simulink model "current_controller_Buck_converter_A01"  (R2025b)
settings: Solver=ode15s  StartTime=0.0  StopTime=0.1  FixedStep=Ts  RelTol=1e-3
values from neighbouring files (symbols this model uses):
  H = -1/(s*R*C)    [type_1_compansator_A01.m]
  R_f = 0.2    [buck_converter_parameters_A01.m]
undefined symbols (not defined in the file or in its folder): ma, Ts
libraries: spsSeriesRLCBranchLib x3, spsCurrentMeasurementLib x2, cstblocks x1, simulink x1, spsDCVoltageSourceLib x1, spsDiodeLib x1, spsMosfetLib x1, spsVoltageMeasurementLib x1, sps_lib x1
settings Model: Creator=arif  LastModifiedBy=arif
settings SolverCC: ZeroCrossAlgorithm=Adaptive
settings DebuggingCC: MaskedZcDiagnostic=none  IgnoredZcDiagnostic=none

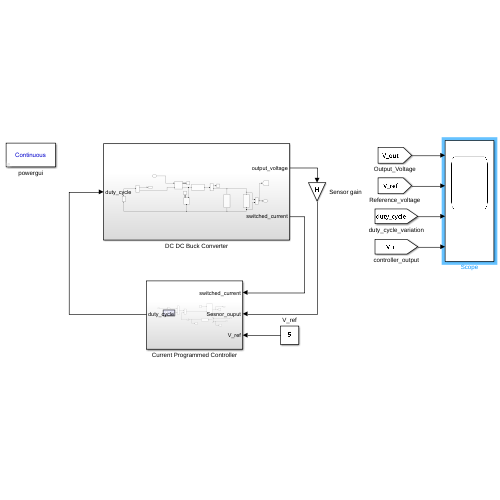
[thumbnail: Simulink's stored preview of the top-level diagram]
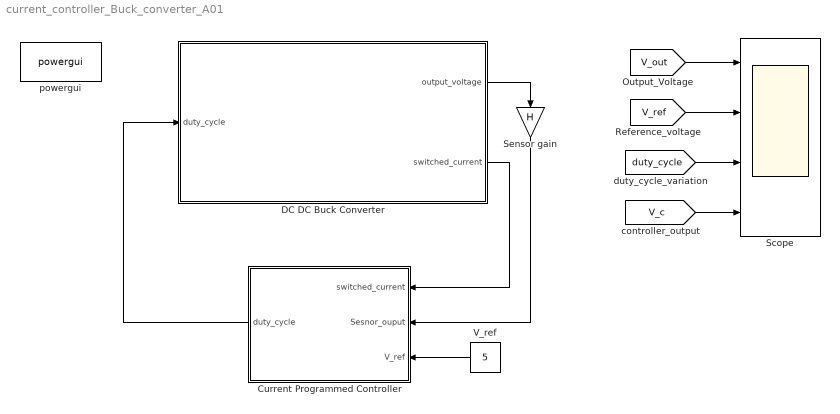
== system current_controller_Buck_converter_A01 ==
  Current Programmed Controller : Subsystem
      settings: PortSchema="{\"entries\":[{\"content\":{\"sides\":[{\"content\":{\"connectorIds\":[\"Out1\"]},\"type\":\"ConnectorPlacement.EquallySpacedRectSide\",\"uuid\":\"f14b5529-64c8-475c-92f8-e2614ee0a8ad\"},{\"content\":{\"connectorIds\":[\"In1\",\"In2\",\"In3\"],\"side\":\"RIGHT\"},\"type\":\"ConnectorPlacement.EquallySpacedRectSide\",\"uuid\":\"ccab92c4-01d4-490c-899e-0d4eb02db195\"},{\"content\":{\"side\":\"TOP\"},\"type\":\"ConnectorPlacement.EquallySpacedRectSide\",\"uuid\":\"b1180856-4250-44ce-8479-d48f19e18262\"}]},\"type\":\"ConnectorPlacement.EquallySpacedConnector\",\"uuid\":\"9f0b6857-1f65-4299-9855-6d8c8b04cf8e\"}],\"packageUris\":[\"http://schema.mathworks.com/mf0/Connector/R2020b\"],\"version\":\"1.0\"}"
  DC DC Buck Converter : Subsystem
  Scope : Scope  NumInputPorts=4
      settings: ActiveDisplayYMinimum=-4.2219957385816729  ActiveDisplayYMaximum=38.006361395242614
  Sensor gain : Gain  Gain=H
  V_ref : Constant  Value=5
  powergui : sps_lib/powergui  Priority=1  SimulationMode=Continuous  SampleTime=50e-6  frequency=60  Iterations=50  frequencyindice=0  Pbase=100e6  ErrMax=1e-4  UnitsV=kV  UnitsW=MW  buscounter=0  FunctionMessages=off  echomessages=off  EnableUseOfTLC=off  CurrentSourceSwitches=off  DisableSnubberDevices=off  DisableRonSwitches=off  DisableVfSwitches=off  DisplayEquations=off  AutomaticDiscreteSolvers=off  SolverType=Tustin/Backward Euler (TBE)  Interpol=off  ExternalGateDelay=off  methode=off  Ts=100  x0status=blocks  SPID=on  SwTol=0  HookPort=off  NonlinearTolerance=1e-4  nMaxIteration=100  ContinueOnMaxIteration=off  RestoreLinks=warning  ResistiveCurrentMeasurement=off  Frange=[0:2:500]  Ylog=off  Xlog=on  ShowGrid=off  save=off  variable=ZData  structure=0  ZoomFFT=off  StartTime=0.0  cycles=1  DisplayStyle=1  fundamental=60  FreqAxis=off  MaxFrequency=1000  frequencyindicesteady=1  RmsSteady=1  display=off
  wires:
  [V_c] -> Scope/4
  [duty_cycle] -> Scope/3
  [V_out] -> Scope/1
  [V_ref] -> Scope/2
  V_ref/1 -> Current Programmed Controller/3(V_ref)
  DC DC Buck Converter/1(output_voltage) -> Sensor gain/1
  Current Programmed Controller/1(duty_cycle) -> DC DC Buck Converter/1(duty_cycle)
  DC DC Buck Converter/2(switched_current) -> Current Programmed Controller/1(switched_current)
  Sensor gain/1 -> Current Programmed Controller/2(Sesnor_ouput)

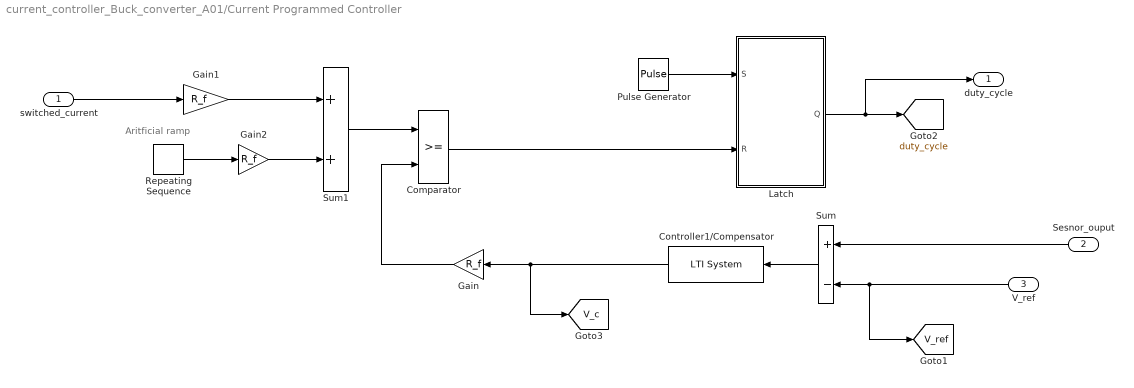
== system current_controller_Buck_converter_A01/Current Programmed Controller ==
  note: Aritficial ramp
  switched_current : Inport
  Sesnor_ouput : Inport  Port=2
  V_ref : Inport  Port=3
  Comparator : RelationalOperator  OutDataTypeStr=boolean  RndMeth=Simplest  InputSameDT=off
  Controller1/Compensator : cstblocks/LTI System  sys=G_PI  IC=[]  PadeOrder=0
  Gain : Gain  Gain=R_f
  Gain1 : Gain  Gain=R_f
  Gain2 : Gain  Gain=R_f
  Latch : Subsystem
  Pulse Generator : DiscretePulseGenerator  PulseType=Time based  Period=Ts  PulseWidth=99
  Repeating Sequence : simulink/Sources/Repeating Sequence  rep_seq_t=[0 Ts]  rep_seq_y=[0 ma*Ts]
  Sum : Sum  Inputs=+-
  Sum1 : Sum
  duty_cycle : Outport
  tag scope: V_c=global, V_ref=global, duty_cycle=global
  wires:
  Gain/1 -> Comparator/2
  switched_current/1 -> Gain1/1
  Sum/1 -> Controller1/Compensator/1
  V_ref/1 -> [V_ref], Sum/2
  Repeating Sequence/1 -> Gain2/1
  Sum1/1 -> Comparator/1
  Gain2/1 -> Sum1/2
  Controller1/Compensator/1 -> [V_c], Gain/1
  Gain1/1 -> Sum1/1
  Latch/1(Q) -> [duty_cycle], duty_cycle/1
  Pulse Generator/1 -> Latch/1(S)
  Comparator/1 -> Latch/2(R)
  Sesnor_ouput/1 -> Sum/1

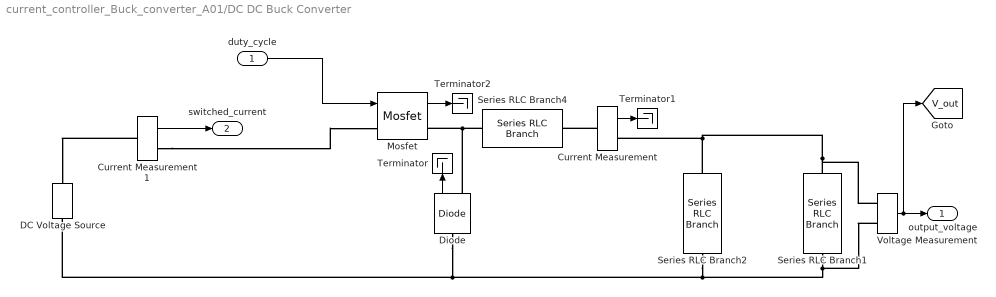
== system current_controller_Buck_converter_A01/DC DC Buck Converter ==
  duty_cycle : Inport
  Current Measurement : spsCurrentMeasurementLib/Current Measurement  PhasorSimulation=off  OutputType=Complex  PSBequivalent=0
  Current Measurement1 : spsCurrentMeasurementLib/Current Measurement  PhasorSimulation=off  OutputType=Complex  PSBequivalent=0
  DC Voltage Source : spsDCVoltageSourceLib/DC Voltage Source  Amplitude=28  Measurements=None
  Diode : spsDiodeLib/Diode  Ron=0.001  Lon=0  Vf=0.8  IC=0  UseSnubber=0  Rs=500  Cs=250e-9  Measurements=on
  Mosfet : spsMosfetLib/Mosfet  Ron=0.1  Lon=0  Rd=0.01  Vfd=0  IC=0  Rs=1e5  Cs=inf  Measurements=on
  Series RLC Branch1 : spsSeriesRLCBranchLib/Series RLC Branch  LConnTagsString=__new0  RConnTagsString=__new0  BranchType=R  Resistance=3  Inductance=1e-3  SetiL0=off  InitialCurrent=0  Capacitance=1e-6  Setx0=off  InitialVoltage=0  Measurements=None
  Series RLC Branch2 : spsSeriesRLCBranchLib/Series RLC Branch  LConnTagsString=__new0  RConnTagsString=__new0  BranchType=C  Resistance=10  Inductance=1e-3  SetiL0=off  InitialCurrent=0  Capacitance=500e-6  Setx0=off  InitialVoltage=0  Measurements=None
  Series RLC Branch4 : spsSeriesRLCBranchLib/Series RLC Branch  LConnTagsString=__new0  RConnTagsString=__new0  BranchType=L  Resistance=10  Inductance=50e-6  SetiL0=off  InitialCurrent=0  Capacitance=1e-6  Setx0=off  InitialVoltage=0  Measurements=None
  Terminator : Terminator
  Terminator1 : Terminator
  Terminator2 : Terminator
  Voltage Measurement : spsVoltageMeasurementLib/Voltage Measurement  PhasorSimulation=off  OutputType=Complex  PSBequivalent=0
  output_voltage : Outport
  switched_current : Outport  Port=2
  tag scope: V_out=global
  wires:
  Current Measurement/1 -> Terminator1/1
  Diode/1 -> Terminator/1
  duty_cycle/1 -> Mosfet/1
  Mosfet/1 -> Terminator2/1
  Current Measurement1/1 -> switched_current/1
  Voltage Measurement/1 -> [V_out], output_voltage/1
  connections:
  Current Measurement1/RConn1 -- Mosfet/LConn1
  Current Measurement1/LConn1 -- DC Voltage Source/RConn1
  Mosfet/RConn1 -- Series RLC Branch4/LConn1 -- Diode/RConn1
  DC Voltage Source/LConn1 -- Series RLC Branch1/RConn1 -- Voltage Measurement/LConn2 -- Series RLC Branch2/RConn1 -- Diode/LConn1
  Series RLC Branch1/LConn1 -- Series RLC Branch2/LConn1 -- Current Measurement/RConn1 -- Voltage Measurement/LConn1
  Current Measurement/LConn1 -- Series RLC Branch4/RConn1

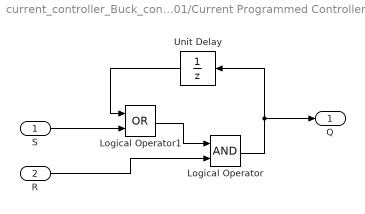
== system current_controller_Buck_converter_A01/Current Programmed Controller/Latch ==
  S : Inport
  R : Inport  Port=2
  Logical Operator : Logic  AllPortsSameDT=off  OutDataTypeStr=boolean
  Logical Operator1 : Logic  Operator=OR  AllPortsSameDT=off  OutDataTypeStr=boolean
  Unit Delay : UnitDelay  SampleTime=-1  HasFrameUpgradeWarning=on
  Q : Outport
  wires:
  Unit Delay/1 -> Logical Operator1/1
  R/1 -> Logical Operator/2
  Logical Operator1/1 -> Logical Operator/1
  Logical Operator/1 -> Q/1, Unit Delay/1
  S/1 -> Logical Operator1/2
